simulink model "half_controlled_rectifier"  (R2024b)
settings: Solver=VariableStepAuto  StartTime=0.0  StopTime=10.0  RelTol=1e-3
undefined symbols (not defined in the file): a
libraries: spsDiodeLib x2, spsThyristorLib x2, spsACVoltageSourceLib x1, spsCurrentMeasurementLib x1, spsDCMachineLib x1, spsDCVoltageSourceLib x1, spsTHDLib x1, spsVoltageMeasurementLib x1, sps_lib x1
settings Model: Creator=lenovo  LastModifiedBy=lenovo
settings DataIOCC: LoggingToFile=on

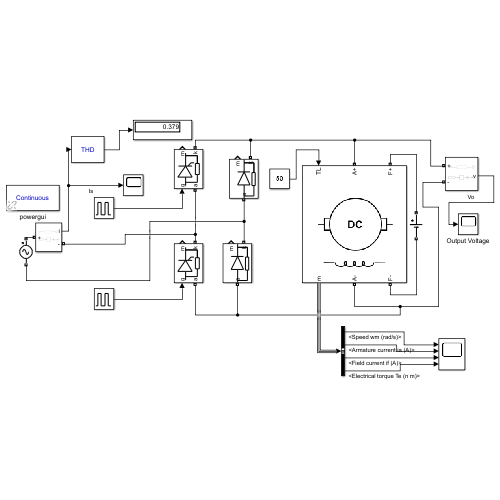
[thumbnail: Simulink's stored preview of the top-level diagram]
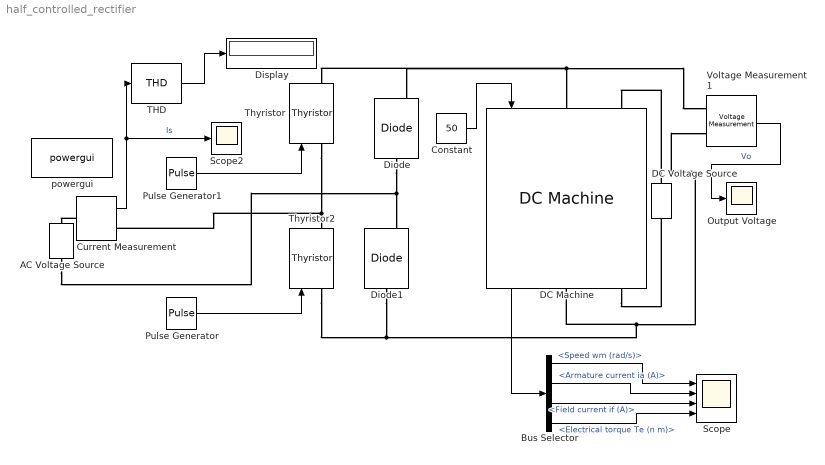
== system half_controlled_rectifier ==
  AC Voltage Source : spsACVoltageSourceLib/AC Voltage Source  Amplitude=230  Phase=0  Frequency=50  SampleTime=0  Measurements=None  BusType=swing  Pref=10e3  Qref=0  Qmin=-inf  Qmax=+inf
  Bus Selector : BusSelector  OutputSignals=Speed wm (rad/s),Armature current ia (A),Field current if (A),Electrical torque Te (n m)
  Constant : Constant  Value=50
  Current Measurement : spsCurrentMeasurementLib/Current Measurement  PhasorSimulation=off  OutputType=Complex  PSBequivalent=0
  DC Machine : spsDCMachineLib/DC Machine  PresetModel=No  MechanicalLoad=Torque TL  FieldType=Wound  ShowDetailedParameters=on  MeasurementBus=off  RLa="[ 0.6  0.012]"  RLf="[ 240  120]"  Laf=1.8  MachineConstant=Torque constant (N.m/A)  Ke=1.8  Kt=1.8  J=1  Bm=0  Tf=0  w0=1  Ifinit=0.916666665761953  TsPowergui=0  TsBlock=-1
  DC Voltage Source : spsDCVoltageSourceLib/DC Voltage Source  Amplitude=220  Measurements=None
  Diode : spsDiodeLib/Diode  Ron=0.001  Lon=0  Vf=0.8  IC=0  UseSnubber=0  Rs=500  Cs=250e-9  Measurements=on
  Diode1 : spsDiodeLib/Diode  Ron=0.001  Lon=0  Vf=0.8  IC=0  UseSnubber=0  Rs=500  Cs=250e-9  Measurements=on
  Display : Display
  Output Voltage : Scope
  Pulse Generator : DiscretePulseGenerator  PulseType=Time based  Period=1/50  PulseWidth=50  PhaseDelay=(a+180)*0.02/360
  Pulse Generator1 : DiscretePulseGenerator  PulseType=Time based  Period=1/50  PulseWidth=50  PhaseDelay=a*0.02/360
  Scope : Scope  NumInputPorts=4
  Scope2 : Scope
  THD : spsTHDLib/THD  Freq=60  Ts=0
  Thyristor : spsThyristorLib/Thyristor  Ron=0.001  Lon=0  Vf=0.8  IC=0  Rs=500  Cs=250e-9  Measurements=on
  Thyristor2 : spsThyristorLib/Thyristor  Ron=0.001  Lon=0  Vf=0.8  IC=0  Rs=500  Cs=250e-9  Measurements=on
  Voltage Measurement1 : spsVoltageMeasurementLib/Voltage Measurement  PhasorSimulation=off  OutputType=Complex  PSBequivalent=0
  powergui : sps_lib/powergui  Priority=1  SimulationMode=Continuous  SampleTime=50e-6  frequency=60  Iterations=50  frequencyindice=50  Pbase=100e6  ErrMax=1e-4  UnitsV=kV  UnitsW=MW  buscounter=0  FunctionMessages=off  echomessages=off  EnableUseOfTLC=off  CurrentSourceSwitches=off  DisableSnubberDevices=off  DisableRonSwitches=off  DisableVfSwitches=off  DisplayEquations=off  AutomaticDiscreteSolvers=off  SolverType=Tustin/Backward Euler (TBE)  Interpol=off  ExternalGateDelay=off  methode=off  Ts=100  x0status=blocks  SPID=on  SwTol=0  HookPort=off  NonlinearTolerance=1e-4  nMaxIteration=100  ContinueOnMaxIteration=off  RestoreLinks=warning  ResistiveCurrentMeasurement=off  Frange=[0:2:500]  Ylog=off  Xlog=on  ShowGrid=off  save=off  variable=ZData  structure=0  ZoomFFT=off  StartTime=0.0  cycles=1  DisplayStyle=1  fundamental=60  FreqAxis=off  MaxFrequency=1000  frequencyindicesteady=1  RmsSteady=1  display=off
  wires:
  THD/1 -> Display/1
  Pulse Generator/1 -> Thyristor2/1
  Pulse Generator1/1 -> Thyristor/1
  Constant/1 -> DC Machine/1
  DC Machine/1 -> Bus Selector/1
  Bus Selector/1 -> Scope/1  "<Speed wm (rad/s)>"
  Bus Selector/2 -> Scope/2  "<Armature current ia (A)>"
  Bus Selector/3 -> Scope/3  "<Field current if (A)>"
  Bus Selector/4 -> Scope/4  "<Electrical torque Te (n m)>"
  Voltage Measurement1/1 -> Output Voltage/1  "Vo"
  Current Measurement/1 -> THD/1, Scope2/1  "Is"
  connections:
  Diode/RConn1 -- Thyristor/RConn1 -- DC Machine/LConn1 -- Voltage Measurement1/LConn1
  Thyristor2/LConn1 -- Diode1/LConn1 -- Voltage Measurement1/LConn2 -- DC Machine/RConn1
  Thyristor/LConn1 -- Current Measurement/RConn1 -- Thyristor2/RConn1
  Current Measurement/LConn1 -- AC Voltage Source/RConn1
  DC Voltage Source/RConn1 -- DC Machine/LConn2
  DC Machine/RConn2 -- DC Voltage Source/LConn1
  Diode/LConn1 -- Diode1/RConn1 -- AC Voltage Source/LConn1
